simulink model "pid_baseline_simulink"  (R2022b)
settings: Solver=ode45  StartTime=0.0  StopTime=30  MaxStep=0.005  RelTol=1e-8  AbsTol=1e-10
settings Model: Creator=邵  LastModifiedBy=邵

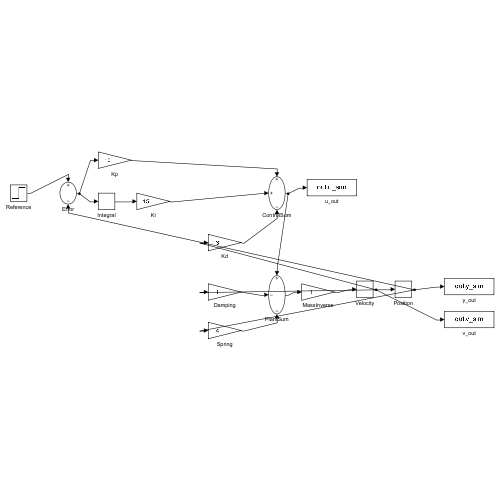
[thumbnail: Simulink's stored preview of the top-level diagram]
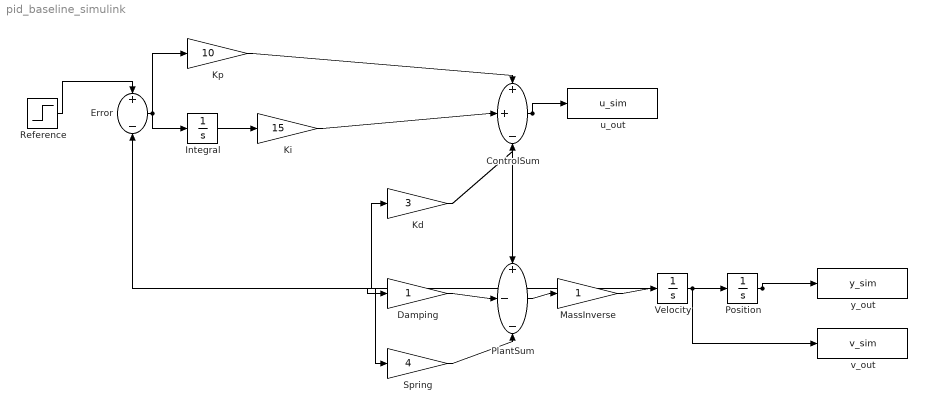
== system pid_baseline_simulink ==
  ControlSum : Sum  Inputs=++-
  Damping : Gain
  Error : Sum  Inputs=+-
  Integral : Integrator
  Kd : Gain  Gain=3
  Ki : Gain  Gain=15
  Kp : Gain  Gain=10
  MassInverse : Gain
  PlantSum : Sum  Inputs=+--
  Position : Integrator
  Reference : Step  Time=0  SampleTime=0
  Spring : Gain  Gain=4
  Velocity : Integrator
  u_out : ToWorkspace  VariableName=u_sim  SaveFormat=Structure With Time  SampleTime=-1
  v_out : ToWorkspace  VariableName=v_sim  SaveFormat=Structure With Time  SampleTime=-1
  y_out : ToWorkspace  VariableName=y_sim  SaveFormat=Structure With Time  SampleTime=-1
  wires:
  Reference/1 -> Error/1
  Position/1 -> Error/2, Spring/1, y_out/1
  Error/1 -> Kp/1, Integral/1
  Integral/1 -> Ki/1
  Kp/1 -> ControlSum/1
  Ki/1 -> ControlSum/2
  Velocity/1 -> Kd/1, Damping/1, Position/1, v_out/1
  Kd/1 -> ControlSum/3
  ControlSum/1 -> u_out/1, PlantSum/1
  Damping/1 -> PlantSum/2
  Spring/1 -> PlantSum/3
  PlantSum/1 -> MassInverse/1
  MassInverse/1 -> Velocity/1
